simulink model "dinamica_booster_23a"  (R2023a)
settings: Solver=VariableStepAuto  StartTime=0.0  StopTime=2  MaxStep=0.001  RelTol=1e-3
values from neighbouring files (symbols this model uses):
  v = linspace(0,60/3.6,100)    [drag_aerodinamico.m]
undefined symbols (not defined in the file or in its folder): dent, drag, force, magnitude
libraries: spsFirstOrderFilterLib x1, eeTransforms x1
settings Model: Creator=USUARIO

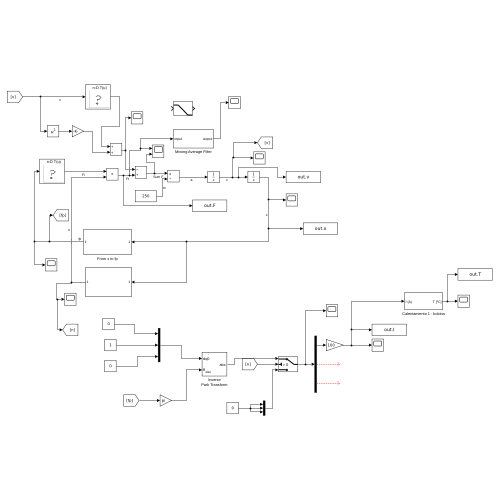
[thumbnail: Simulink's stored preview of the top-level diagram]
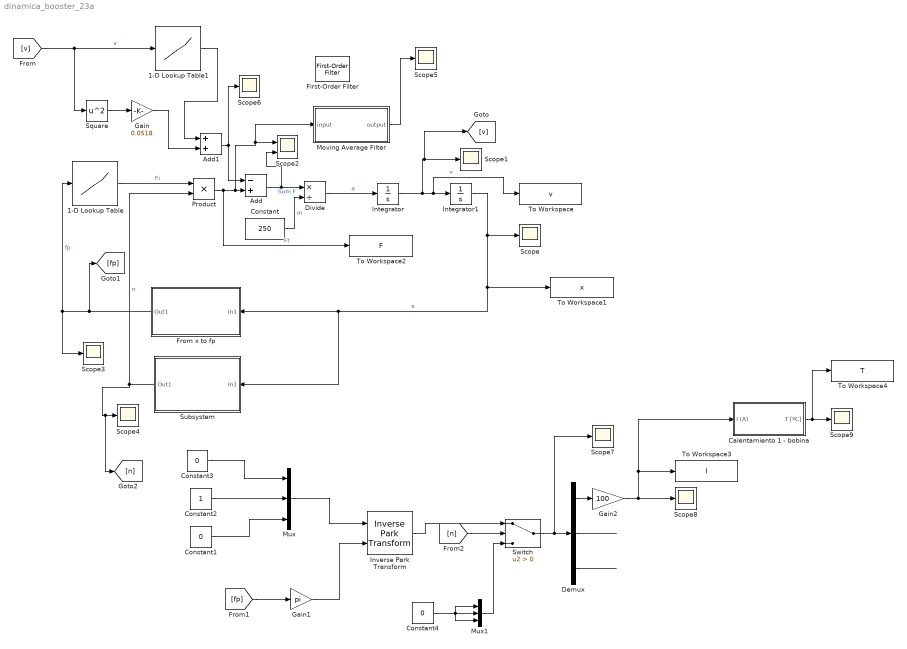
== system dinamica_booster_23a ==
  1-D Lookup Table : Lookup_n-D  NumberOfTableDimensions=1  BreakpointsForDimension1=dent  Table=force  InternalRulePriority=Speed  RndMeth=Simplest
  1-D Lookup Table1 : Lookup_n-D  NumberOfTableDimensions=1  BreakpointsForDimension1=v  Table=drag  InternalRulePriority=Speed  RndMeth=Simplest
  Add : Sum  Inputs=-+
  Add1 : Sum
  Calentamiento 1 - bobina : Subsystem
  Constant : Constant  Value=250
  Constant1 : Constant  Value=0
  Constant2 : Constant
  Constant3 : Constant  Value=0
  Constant4 : Constant  Value=0
  Demux : Demux  Outputs=3
  Divide : Product  Inputs=*/
  First-Order Filter : spsFirstOrderFilterLib/First-Order Filter  FilterType=Lowpass  Tc=10e-3  Ts=0  Initialize=on  Vac_Init=[0, 0, 60]  Vdc_Init=0  PlotResponse=off  FreqRange="[0,  200,  1]"
  From x to fp : Subsystem
  Gain : Gain  Gain=0.0518
  Gain1 : Gain  Gain=pi
  Gain2 : Gain  Gain=100
  Integrator : Integrator  InitialCondition=1
  Integrator1 : Integrator
  Inverse Park Transform : eeTransforms/Inverse Park Transform  AxisAlignment=Q-axis  PowerInvariant=off
      settings: LibrarySourceBlock=|
      | ee_sl_lib/Mathematical
      | Transforms/Inverse
      | Park Transform
  Moving Average Filter : Subsystem  mask{M=50, fs=-1}
      mask prompts: M "Orden del filtro (M)"; fs "Frecuencia de muestreo (fs)"
  Mux : Mux  Inputs=3
  Mux1 : Mux  Inputs=3
  Product : Product
  Scope{,1,3..9} (9 alike) : Scope
  Scope2 : Scope  NumInputPorts=2
  Square : Math  Operator=square
  Subsystem : Subsystem
  Switch : Switch  Criteria=u2 > Threshold  SaturateOnIntegerOverflow=off  InputSameDT=off
  To Workspace : ToWorkspace  VariableName=v  SaveFormat=Timeseries  SampleTime=-1
  To Workspace1 : ToWorkspace  VariableName=x  SaveFormat=Timeseries  SampleTime=-1
  To Workspace2 : ToWorkspace  VariableName=F  SaveFormat=Timeseries  SampleTime=-1
  To Workspace3 : ToWorkspace  VariableName=I  SaveFormat=Timeseries  SampleTime=-1
  To Workspace4 : ToWorkspace  VariableName=T  SaveFormat=Timeseries  SampleTime=-1
  wires:
  1-D Lookup Table/1 -> Product/1  "Fi"
  Subsystem/1(Out1) -> Product/2, [n], Scope4/1  "n"
  Product/1 -> To Workspace2/1, Moving Average Filter/1(input), Scope2/1, Add/2  "Ft"
  Constant/1 -> Divide/2  "m"
  Divide/1 -> Integrator/1  "a"
  [v] -> Square/1, 1-D Lookup Table1/1  "v"
  1-D Lookup Table1/1 -> Add1/1
  Square/1 -> Gain/1
  Add1/1 -> Add/1, Scope6/1
  Gain/1 -> Add1/2
  Add/1 -> Scope2/2, Divide/1  "Sum F"
  Integrator/1 -> [v], Scope1/1, To Workspace/1, Integrator1/1  "v"
  Integrator1/1 -> Scope/1, Subsystem/1(In1), From x to fp/1(In1), To Workspace1/1  "x"
  From x to fp/1(Out1) -> [fp], 1-D Lookup Table/1, Scope3/1  "fp"
  Moving Average Filter/1(output) -> Scope5/1
  [fp] -> Gain1/1
  Inverse Park Transform/1 -> Switch/1
  Demux/3 -> ?
  Constant1/1 -> Mux/3
  Mux/1 -> Inverse Park Transform/1
  Demux/1 -> Gain2/1
  Gain1/1 -> Inverse Park Transform/2
  Constant3/1 -> Mux/1
  Demux/2 -> ?
  Constant2/1 -> Mux/2
  [n] -> Switch/2
  Switch/1 -> Scope7/1, Demux/1
  Constant4/1 -> Mux1/3, Mux1/1, Mux1/2
  Mux1/1 -> Switch/3
  Calentamiento 1 - bobina/1(T [ºC]) -> To Workspace4/1, Scope9/1
  Gain2/1 -> Calentamiento 1 - bobina/1(I (A)), To Workspace3/1, Scope8/1

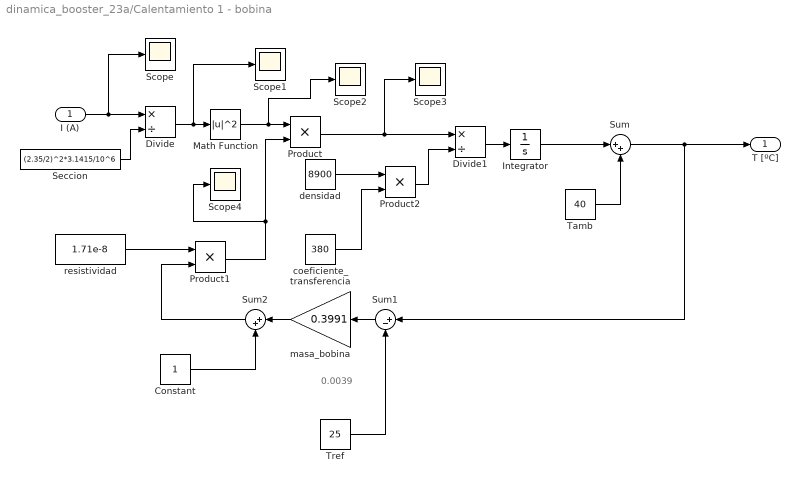
== system dinamica_booster_23a/Calentamiento 1 - bobina ==
  note: 0.0039
  I (A) : Inport
  Constant : Constant
  Divide : Product  Inputs=*/
  Divide1 : Product  Inputs=*/
  Integrator : Integrator
  Math Function : Math  Operator=magnitude^2
  Product : Product
  Product1 : Product
  Product2 : Product
  Scope{,1..4} (5 alike) : Scope
  Seccion : Constant  Value=(2.35/2)^2*3.1415/10^6
  Sum : Sum  Inputs=|++
  Sum1 : Sum  Inputs=|+-
  Sum2 : Sum  Inputs=|++
  Tamb : Constant  Value=40
  Tref : Constant  Value=25
  coeficiente_transferencia : Constant  Value=380
  densidad : Constant  Value=8900
  masa_bobina : Gain  Gain=0.3991
  resistividad : Constant  Value=1.71e-8
  T [ºC] : Outport
  wires:
  I (A)/1 -> Scope/1, Divide/1
  Seccion/1 -> Divide/2
  Divide/1 -> Scope1/1, Math Function/1
  Math Function/1 -> Scope2/1, Product/1
  Product/1 -> Scope3/1, Divide1/1
  Divide1/1 -> Integrator/1
  Integrator/1 -> Sum/1
  Tamb/1 -> Sum/2
  Sum/1 -> Sum1/1, T [ºC]/1
  Sum1/1 -> masa_bobina/1
  Tref/1 -> Sum1/2
  masa_bobina/1 -> Sum2/1
  Constant/1 -> Sum2/2
  resistividad/1 -> Product1/1
  Sum2/1 -> Product1/2
  Product1/1 -> Scope4/1, Product/2
  Product2/1 -> Divide1/2
  densidad/1 -> Product2/1
  coeficiente_transferencia/1 -> Product2/2

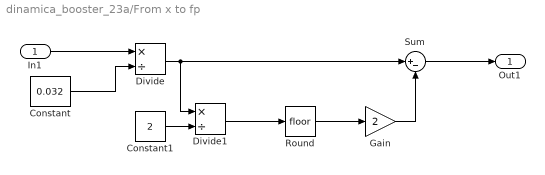
== system dinamica_booster_23a/From x to fp ==
  In1 : Inport
  Constant : Constant  Value=0.032
  Constant1 : Constant  Value=2
  Divide : Product  Inputs=*/
  Divide1 : Product  Inputs=*/
  Gain : Gain  Gain=2
  Round : Rounding
  Sum : Sum  Inputs=|+-
  Out1 : Outport
  wires:
  In1/1 -> Divide/1
  Constant/1 -> Divide/2
  Divide/1 -> Divide1/1, Sum/1
  Divide1/1 -> Round/1
  Round/1 -> Gain/1
  Constant1/1 -> Divide1/2
  Gain/1 -> Sum/2
  Sum/1 -> Out1/1

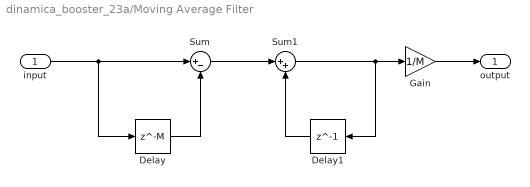
== system dinamica_booster_23a/Moving Average Filter ==
  input : Inport
  Delay : Delay  DelayLength=M  SampleTime=fs
  Delay1 : Delay  DelayLength=1  SampleTime=fs
  Gain : Gain  Gain=1/M
  Sum : Sum  Inputs=|+-
  Sum1 : Sum  Inputs=|++
  output : Outport
  wires:
  input/1 -> Delay/1, Sum/1
  Delay/1 -> Sum/2
  Sum/1 -> Sum1/1
  Sum1/1 -> Delay1/1, Gain/1
  Delay1/1 -> Sum1/2
  Gain/1 -> output/1

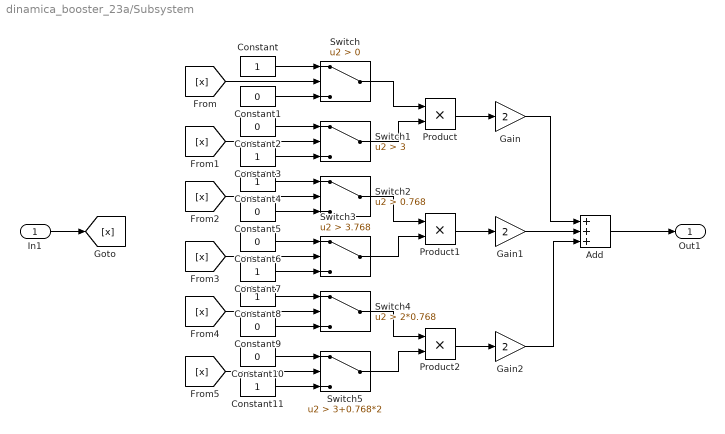
== system dinamica_booster_23a/Subsystem ==
  In1 : Inport
  Add : Sum  Inputs=+++
  Constant{,3..4,7..8,11} (6 alike) : Constant
  Constant{1..2,5..6,9..10} (6 alike) : Constant  Value=0
  Gain : Gain  Gain=2
  Gain1 : Gain  Gain=2
  Gain2 : Gain  Gain=2
  Product : Product
  Product1 : Product
  Product2 : Product
  Switch : Switch  Criteria=u2 > Threshold  SaturateOnIntegerOverflow=off  InputSameDT=off
  Switch1 : Switch  Criteria=u2 > Threshold  Threshold=3  SaturateOnIntegerOverflow=off  InputSameDT=off
  Switch2 : Switch  Criteria=u2 > Threshold  Threshold=0.768  SaturateOnIntegerOverflow=off  InputSameDT=off
  Switch3 : Switch  Criteria=u2 > Threshold  Threshold=3.768  SaturateOnIntegerOverflow=off  InputSameDT=off
  Switch4 : Switch  Criteria=u2 > Threshold  Threshold=2*0.768  SaturateOnIntegerOverflow=off  InputSameDT=off
  Switch5 : Switch  Criteria=u2 > Threshold  Threshold=3+0.768*2  SaturateOnIntegerOverflow=off  InputSameDT=off
  Out1 : Outport
  wires:
  In1/1 -> [x]
  Add/1 -> Out1/1
  Product/1 -> Gain/1
  Constant1/1 -> Switch/3
  Switch/1 -> Product/1
  Product2/1 -> Gain2/1
  Gain1/1 -> Add/2
  [x] -> Switch/2
  Constant2/1 -> Switch1/1
  [x] -> Switch1/2
  Constant/1 -> Switch/1
  Switch5/1 -> Product2/2
  Switch1/1 -> Product/2
  Switch3/1 -> Product1/2
  Switch2/1 -> Product1/1
  Constant10/1 -> Switch5/1
  [x] -> Switch5/2
  Constant11/1 -> Switch5/3
  Gain/1 -> Add/1
  Product1/1 -> Gain1/1
  [x] -> Switch3/2
  Gain2/1 -> Add/3
  [x] -> Switch2/2
  Constant8/1 -> Switch4/1
  Constant6/1 -> Switch3/1
  Constant9/1 -> Switch4/3
  Constant3/1 -> Switch1/3
  Constant4/1 -> Switch2/1
  Constant7/1 -> Switch3/3
  Constant5/1 -> Switch2/3
  [x] -> Switch4/2
  Switch4/1 -> Product2/1
